simulink model "solar_tracker_plant"  (R2026b)
settings: Solver=ode4  StopTime=60  FixedStep=0.01
model workspace (MAT data in the model file):
  targetAzimuthInput = timeseries
  targetAzimuthInput.Name = 'unnamed'
  targetAzimuthInput.DataInfo = tsdata.datametadata
  targetAzimuthInput.DataInfo.Interpolation = tsdata.interpolation
  targetAzimuthInput.DataInfo.Interpolation.Fhandle : function handle (value not decoded)
  targetAzimuthInput.DataInfo.Interpolation.Name = 'linear'
  targetAzimuthInput.TimeInfo = tsdata.timemetadata
  targetAzimuthInput.TimeInfo.Length = 2
  targetAzimuthInput.TimeInfo.DuplicateTimes = 0
  targetAzimuthInput.TimeInfo.Time_ = [0; 86400]
  targetAzimuthInput.TimeInfo.Initialized = 1
  targetAzimuthInput.QualityInfo = tsdata.qualmetadata
  targetAzimuthInput.Data_ = [0; 0]
  targetTiltInput = timeseries
  targetTiltInput.Name = 'unnamed'
  targetTiltInput.DataInfo = tsdata.datametadata
  targetTiltInput.DataInfo.Interpolation = tsdata.interpolation
  targetTiltInput.DataInfo.Interpolation.Fhandle : function handle (value not decoded)
  targetTiltInput.DataInfo.Interpolation.Name = 'linear'
  targetTiltInput.TimeInfo = tsdata.timemetadata
  targetTiltInput.TimeInfo.Length = 2
  targetTiltInput.TimeInfo.DuplicateTimes = 0
  targetTiltInput.TimeInfo.Time_ = [0; 86400]
  targetTiltInput.TimeInfo.Initialized = 1
  targetTiltInput.QualityInfo = tsdata.qualmetadata
  targetTiltInput.Data_ = [0; 0]
libraries: fl_lib x22, nesl_utility x16, sl_discontinuities x2
settings Model: Creator=Jhons Janner Samuel  LastModifiedBy=Jhons Janner Samuel
settings SimscapeCC: SimscapeLogType=all  SimscapeNominalValues="[{\"value\":\"1\",\"unit\":\"A\"},{\"value\":\"1\",\"unit\":\"bar\"},{\"value\":\"1\",\"unit\":\"cm^2\"},{\"value\":\"1\",\"unit\":\"cm^3/s\"},{\"value\":\"1\",\"unit\":\"kJ/kg\"},{\"value\":\"1\",\"unit\":\"kW\"},{\"value\":\"1\",\"unit\":\"l\"},{\"value\":\"1\",\"unit\":\"N\"},{\"value\":\"1\",\"unit\":\"N*m\"},{\"value\":\"1\",\"unit\":\"V\"},{\"value\":\"0.001\",\"unit\":\"Wb\"}]"  SimscapeUseEnergyAccounting=off

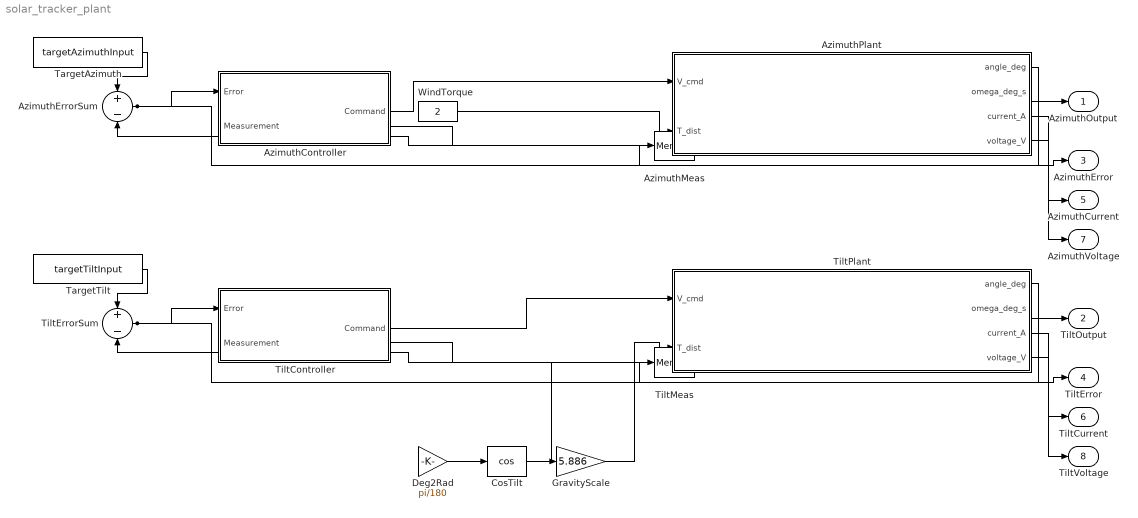
== system solar_tracker_plant ==
  AzimuthController : Subsystem
  AzimuthErrorSum : Sum  Inputs=+-
  AzimuthMeas : Memory
  AzimuthPlant : Subsystem
  CosTilt : Trigonometry  Operator=cos
  Deg2Rad : Gain  Gain=pi/180
  GravityScale : Gain  Gain=5.886
  TargetAzimuth : FromWorkspace  VariableName=targetAzimuthInput
  TargetTilt : FromWorkspace  VariableName=targetTiltInput
  TiltController : Subsystem
  TiltErrorSum : Sum  Inputs=+-
  TiltMeas : Memory
  TiltPlant : Subsystem
  WindTorque : Constant  Value=2
  AzimuthOutput : Outport
  TiltOutput : Outport  Port=2
  AzimuthError : Outport  Port=3
  TiltError : Outport  Port=4
  AzimuthCurrent : Outport  Port=5
  TiltCurrent : Outport  Port=6
  AzimuthVoltage : Outport  Port=7
  TiltVoltage : Outport  Port=8
  wires:
  TargetAzimuth/1 -> AzimuthErrorSum/1
  TargetTilt/1 -> TiltErrorSum/1
  TiltMeas/1 -> Deg2Rad/1, TiltOutput/1, TiltErrorSum/2, TiltController/2(Measurement)
  Deg2Rad/1 -> CosTilt/1
  CosTilt/1 -> GravityScale/1
  AzimuthErrorSum/1 -> AzimuthController/1(Error), AzimuthError/1
  AzimuthController/1(Command) -> AzimuthPlant/1(V_cmd)
  AzimuthPlant/1(angle_deg) -> AzimuthMeas/1
  AzimuthMeas/1 -> AzimuthOutput/1, AzimuthErrorSum/2, AzimuthController/2(Measurement)
  TiltErrorSum/1 -> TiltController/1(Error), TiltError/1
  TiltController/1(Command) -> TiltPlant/1(V_cmd)
  TiltPlant/1(angle_deg) -> TiltMeas/1
  AzimuthPlant/3(current_A) -> AzimuthCurrent/1
  TiltPlant/3(current_A) -> TiltCurrent/1
  AzimuthPlant/4(voltage_V) -> AzimuthVoltage/1
  TiltPlant/4(voltage_V) -> TiltVoltage/1
  WindTorque/1 -> AzimuthPlant/2(T_dist)
  GravityScale/1 -> TiltPlant/2(T_dist)

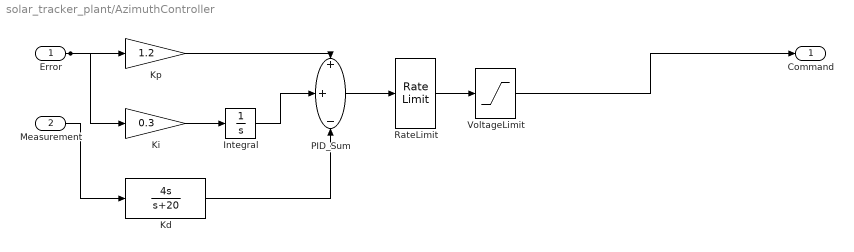
== system solar_tracker_plant/AzimuthController ==
  Error : Inport
  Measurement : Inport  Port=2
  Integral : Integrator  LimitOutput=on  UpperSaturationLimit=80  LowerSaturationLimit=-80
  Kd : TransferFcn  Numerator=[4 0]  Denominator=[1 20]
  Ki : Gain  Gain=0.3
  Kp : Gain  Gain=1.2
  PID_Sum : Sum  Inputs=++-
  RateLimit : RateLimiter  RisingSlewLimit=2400  FallingSlewLimit=-2400  SampleTimeMode=inherited
  VoltageLimit : Saturate  UpperLimit=24  LowerLimit=-24
  Command : Outport
  wires:
  Error/1 -> Kp/1, Ki/1
  Ki/1 -> Integral/1
  Measurement/1 -> Kd/1
  Kp/1 -> PID_Sum/1
  Integral/1 -> PID_Sum/2
  Kd/1 -> PID_Sum/3
  PID_Sum/1 -> RateLimit/1
  RateLimit/1 -> VoltageLimit/1
  VoltageLimit/1 -> Command/1

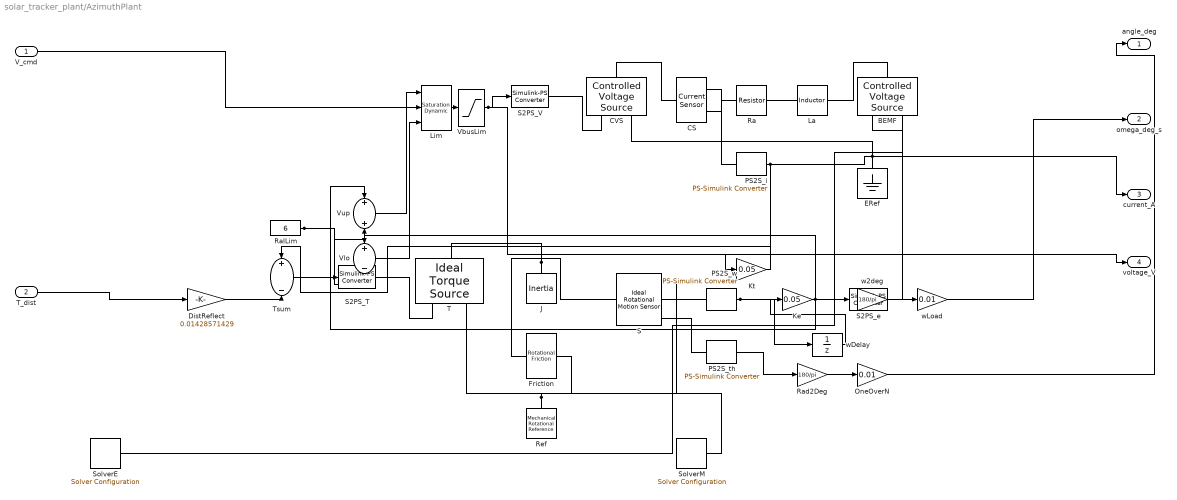
== system solar_tracker_plant/AzimuthPlant ==
  V_cmd : Inport
  T_dist : Inport  Port=2
  BEMF : fl_lib/Electrical/Electrical Sources/Controlled Voltage Source
  CS : fl_lib/Electrical/Electrical Sensors/Current Sensor
  CVS : fl_lib/Electrical/Electrical Sources/Controlled Voltage Source
  DistReflect : Gain  Gain=0.01428571429
  ERef : fl_lib/Electrical/Electrical Elements/Electrical Reference
  Friction : fl_lib/Mechanical/Rotational Elements/Rotational Friction  brkwy_trq=0.01 N*m  brkwy_vel=0.01 rad/s  Col_trq=0.01 N*m  visc_coef=0.0001 N*m*s/rad  w_specify=off  w_priority=None  w=0 rad/s  w_nominal_specify=off  w_nominal_value=1  w_nominal_unit=rad/s  t_specify=off  t_priority=None  t=0 N*m  t_nominal_specify=off  t_nominal_value=1  t_nominal_unit=N*m
  J : fl_lib/Mechanical/Rotational Elements/Inertia  inertia=0.00081 kg*m^2  num_ports=foundation.enum.numPorts2.one  w_specify=off  w_priority=High  w=0 rad/s  w_nominal_specify=off  w_nominal_value=1  w_nominal_unit=rad/s  t_specify=off  t_priority=None  t=0 N*m  t_nominal_specify=off  t_nominal_value=1  t_nominal_unit=N*m
  Ke : Gain  Gain=0.05
  Kt : Gain  Gain=0.05
  La : fl_lib/Electrical/Electrical Elements/Inductor  l=0.0005 H  r=0 Ohm  g=1e-9 1/Ohm  i_specify=off  i_priority=None  i=0 A  i_nominal_specify=off  i_nominal_value=1  i_nominal_unit=A  v_specify=off  v_priority=None  v=0 V  v_nominal_specify=off  v_nominal_value=1  v_nominal_unit=V  i_L_specify=off  i_L_priority=High  i_L=0 A  i_L_nominal_specify=off  i_L_nominal_value=1  i_L_nominal_unit=A
  Lim : sl_discontinuities/Saturation Dynamic  OutMin=[]  OutMax=[]  OutDataTypeStr=Inherit: Same as second input  OutDataType=fixdt(1, 16)  OutScaling=2^-10  DoSatur=off
      settings: LibrarySourceBlock=|
      | simulink/Discontinuities/Saturation
      | Dynamic
  OneOverN : Gain  Gain=0.01
  PS2S_i : nesl_utility/PS-Simulink Converter  PhysicalDomain=network_engine_domain  SubClassName=ps_output  LeftPortType=input  RightPortType=output  PseudoPeriodic=off  Frequencies=[]  VectorFormat=inherit  Unit=inherit  AffineConversion=off
  PS2S_th : nesl_utility/PS-Simulink Converter  PhysicalDomain=network_engine_domain  SubClassName=ps_output  LeftPortType=input  RightPortType=output  PseudoPeriodic=off  Frequencies=[]  VectorFormat=inherit  Unit=inherit  AffineConversion=off
  PS2S_w : nesl_utility/PS-Simulink Converter  PhysicalDomain=network_engine_domain  SubClassName=ps_output  LeftPortType=input  RightPortType=output  PseudoPeriodic=off  Frequencies=[]  VectorFormat=inherit  Unit=inherit  AffineConversion=off
  Ra : fl_lib/Electrical/Electrical Elements/Resistor  R=1.2 Ohm  i_specify=off  i_priority=None  i=0 A  i_nominal_specify=off  i_nominal_value=1  i_nominal_unit=A  v_specify=off  v_priority=None  v=0 V  v_nominal_specify=off  v_nominal_value=1  v_nominal_unit=V
  RaILim : Constant  Value=6
  Rad2Deg : Gain  Gain=180/pi
  Ref : fl_lib/Mechanical/Rotational Elements/Mechanical Rotational Reference
  S : fl_lib/Mechanical/Mechanical Sensors/Ideal Rotational Motion Sensor  reference=foundation.enum.MeasurementReference.difference  acceleration_port=false  velocity_port=true  position_port=true  wrap_angle=false  offset=0 rad
  S2PS_T : nesl_utility/Simulink-PS Converter  PhysicalDomain=network_engine_domain  SubClassName=ps_input  LeftPortType=input  RightPortType=output  PseudoPeriodic=off  Frequencies=[]  NoiseDistribution=none  NoiseParameters=[]  Unit=1  AffineConversion=off  FilteringAndDerivatives=provide  SimscapeFilterOrder=1  InputFilterTimeConstant=0.001  UdotUserProvided=0
  S2PS_V : nesl_utility/Simulink-PS Converter  PhysicalDomain=network_engine_domain  SubClassName=ps_input  LeftPortType=input  RightPortType=output  PseudoPeriodic=off  Frequencies=[]  NoiseDistribution=none  NoiseParameters=[]  Unit=1  AffineConversion=off  FilteringAndDerivatives=provide  SimscapeFilterOrder=1  InputFilterTimeConstant=0.001  UdotUserProvided=0
  S2PS_e : nesl_utility/Simulink-PS Converter  PhysicalDomain=network_engine_domain  SubClassName=ps_input  LeftPortType=input  RightPortType=output  PseudoPeriodic=off  Frequencies=[]  NoiseDistribution=none  NoiseParameters=[]  Unit=1  AffineConversion=off  FilteringAndDerivatives=provide  SimscapeFilterOrder=1  InputFilterTimeConstant=0.001  UdotUserProvided=0
  SolverE : nesl_utility/Solver Configuration  PhysicalDomain=network_engine_domain  SubClassName=solver  LeftPortType=input  RightPortType=generic  Tones=[]  Harmonics=[]  SimulateNoise=off  Profile=off  UseLocalSampling=off  EnableSwitchedLinearOptims=on  FrequencyDomain=off  UseCCode=off  RelTol=0.001  AbsTol=0.001  MinStep=1e-09  ToWorkspace=off  RevertToSquareIcSolve=off  NumHomotopyIterations=100  PhasorMode=off  PhasorModeNumHarmonics=1  ConsistencySolver=NEWTON_XTOL_AFTER_FTOL  CanonicalOrdering=CANONICAL  OptimizeIntermediates=OPTIMIZED  MulticoreSolverChoice=BACKWARD_EULER  IndexReductionMethod=DerivativeReplacement  DoDC=off  ResidualTolerance=1e-09  ConsistencyTolSource=GLOBAL  ConsistencyAbsTol=0.001  ConsistencyRelTol=0.001  ConsistencyTolFactor=0.001  UseLocalSolver=on  LocalSolverChoice=NE_BACKWARD_EULER_ADVANCER  ResolveIndetEquations=on  FunctionEvalNumThread=1  LocalSolverSampleTime=0.01  DoFixedCost=off  MaxNonlinIter=3  MaxModeIter=2  ComputeImpulses=off  ImpulseIterations=2  LinearAlgebra=auto  LinearAlgebraNumThread=0  EquationFormulation=NE_TIME_EF  DelaysMemoryBudget=1024  AutomaticFiltering=on  FilteringTimeConstant=0.001  PartitionStorageMethod=AS_NEEDED  PartitionMemoryBudget=1024  PartitionMethod=BALANCED  MultibodyUseLocalSolver=off  MultibodyLocalSolverChoice=ODE1  MultibodyLocalSolverSampleTime=0.001
  SolverM : nesl_utility/Solver Configuration  PhysicalDomain=network_engine_domain  SubClassName=solver  LeftPortType=input  RightPortType=generic  Tones=[]  Harmonics=[]  SimulateNoise=off  Profile=off  UseLocalSampling=off  EnableSwitchedLinearOptims=on  FrequencyDomain=off  UseCCode=off  RelTol=0.001  AbsTol=0.001  MinStep=1e-09  ToWorkspace=off  RevertToSquareIcSolve=off  NumHomotopyIterations=100  PhasorMode=off  PhasorModeNumHarmonics=1  ConsistencySolver=NEWTON_XTOL_AFTER_FTOL  CanonicalOrdering=CANONICAL  OptimizeIntermediates=OPTIMIZED  MulticoreSolverChoice=BACKWARD_EULER  IndexReductionMethod=DerivativeReplacement  DoDC=off  ResidualTolerance=1e-09  ConsistencyTolSource=GLOBAL  ConsistencyAbsTol=0.001  ConsistencyRelTol=0.001  ConsistencyTolFactor=0.001  UseLocalSolver=on  LocalSolverChoice=NE_BACKWARD_EULER_ADVANCER  ResolveIndetEquations=on  FunctionEvalNumThread=1  LocalSolverSampleTime=0.01  DoFixedCost=off  MaxNonlinIter=3  MaxModeIter=2  ComputeImpulses=off  ImpulseIterations=2  LinearAlgebra=auto  LinearAlgebraNumThread=0  EquationFormulation=NE_TIME_EF  DelaysMemoryBudget=1024  AutomaticFiltering=on  FilteringTimeConstant=0.001  PartitionStorageMethod=AS_NEEDED  PartitionMemoryBudget=1024  PartitionMethod=BALANCED  MultibodyUseLocalSolver=off  MultibodyLocalSolverChoice=ODE1  MultibodyLocalSolverSampleTime=0.001
  T : fl_lib/Mechanical/Mechanical Sources/Ideal Torque Source
  Tsum : Sum  Inputs=+-
  VbusLim : Saturate  UpperLimit=24  LowerLimit=-24
  Vlo : Sum  Inputs=+-
  Vup : Sum
  w2deg : Gain  Gain=180/pi
  wDelay : UnitDelay  SampleTime=0.01
  wLoad : Gain  Gain=0.01
  angle_deg : Outport
  omega_deg_s : Outport  Port=2
  current_A : Outport  Port=3
  voltage_V : Outport  Port=4
  wires:
  V_cmd/1 -> Lim/2
  Vup/1 -> Lim/1
  Vlo/1 -> Lim/3
  Lim/1 -> VbusLim/1
  VbusLim/1 -> S2PS_V/1, voltage_V/1
  Ke/1 -> Vup/1, Vlo/1, S2PS_e/1
  RaILim/1 -> Vup/2, Vlo/2
  PS2S_i/1 -> Kt/1, current_A/1
  Kt/1 -> Tsum/1
  T_dist/1 -> DistReflect/1
  DistReflect/1 -> Tsum/2
  Tsum/1 -> S2PS_T/1
  PS2S_w/1 -> wDelay/1, w2deg/1
  wDelay/1 -> Ke/1
  w2deg/1 -> wLoad/1
  wLoad/1 -> omega_deg_s/1
  PS2S_th/1 -> Rad2Deg/1
  Rad2Deg/1 -> OneOverN/1
  OneOverN/1 -> angle_deg/1
  connections:
  CS/RConn1 -- PS2S_i/LConn1
  S2PS_V/RConn1 -- CVS/RConn1
  S2PS_e/RConn1 -- BEMF/RConn1
  S2PS_T/RConn1 -- T/RConn1
  CVS/LConn1 -- CS/LConn1
  CS/RConn2 -- Ra/LConn1
  Ra/RConn1 -- La/LConn1
  La/RConn1 -- BEMF/LConn1
  BEMF/RConn2 -- CVS/RConn2 -- ERef/LConn1 -- SolverE/RConn1
  T/LConn1 -- Friction/LConn1 -- J/LConn1 -- S/LConn1
  Friction/RConn1 -- T/RConn2 -- S/RConn1 -- Ref/LConn1 -- SolverM/RConn1
  S/RConn2 -- PS2S_w/LConn1
  S/RConn3 -- PS2S_th/LConn1

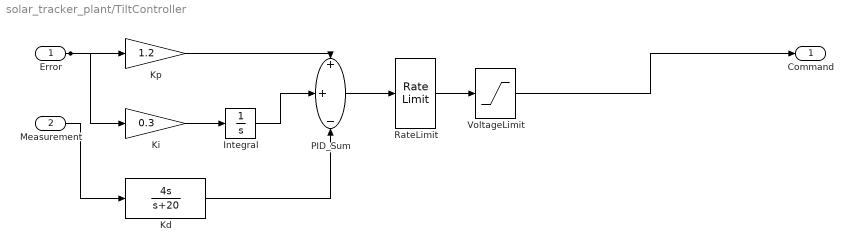
== system solar_tracker_plant/TiltController ==
  Error : Inport
  Measurement : Inport  Port=2
  Integral : Integrator  LimitOutput=on  UpperSaturationLimit=80  LowerSaturationLimit=-80
  Kd : TransferFcn  Numerator=[4 0]  Denominator=[1 20]
  Ki : Gain  Gain=0.3
  Kp : Gain  Gain=1.2
  PID_Sum : Sum  Inputs=++-
  RateLimit : RateLimiter  RisingSlewLimit=2400  FallingSlewLimit=-2400  SampleTimeMode=inherited
  VoltageLimit : Saturate  UpperLimit=24  LowerLimit=-24
  Command : Outport
  wires:
  Error/1 -> Kp/1, Ki/1
  Ki/1 -> Integral/1
  Measurement/1 -> Kd/1
  Kp/1 -> PID_Sum/1
  Integral/1 -> PID_Sum/2
  Kd/1 -> PID_Sum/3
  PID_Sum/1 -> RateLimit/1
  RateLimit/1 -> VoltageLimit/1
  VoltageLimit/1 -> Command/1

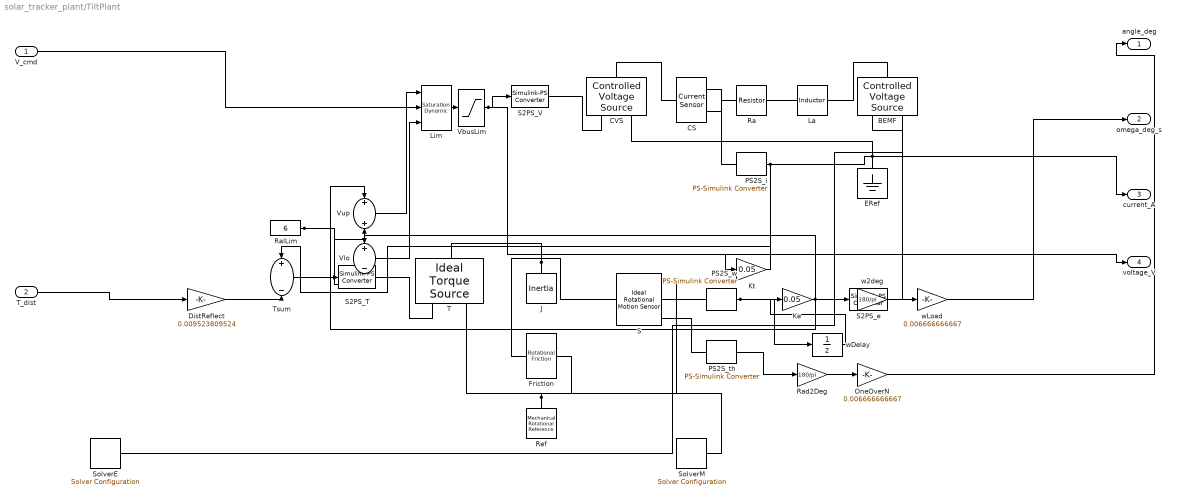
== system solar_tracker_plant/TiltPlant ==
  V_cmd : Inport
  T_dist : Inport  Port=2
  BEMF : fl_lib/Electrical/Electrical Sources/Controlled Voltage Source
  CS : fl_lib/Electrical/Electrical Sensors/Current Sensor
  CVS : fl_lib/Electrical/Electrical Sources/Controlled Voltage Source
  DistReflect : Gain  Gain=0.009523809524
  ERef : fl_lib/Electrical/Electrical Elements/Electrical Reference
  Friction : fl_lib/Mechanical/Rotational Elements/Rotational Friction  brkwy_trq=0.01 N*m  brkwy_vel=0.01 rad/s  Col_trq=0.01 N*m  visc_coef=0.0001 N*m*s/rad  w_specify=off  w_priority=None  w=0 rad/s  w_nominal_specify=off  w_nominal_value=1  w_nominal_unit=rad/s  t_specify=off  t_priority=None  t=0 N*m  t_nominal_specify=off  t_nominal_value=1  t_nominal_unit=N*m
  J : fl_lib/Mechanical/Rotational Elements/Inertia  inertia=0.0001655555556 kg*m^2  num_ports=foundation.enum.numPorts2.one  w_specify=off  w_priority=High  w=0 rad/s  w_nominal_specify=off  w_nominal_value=1  w_nominal_unit=rad/s  t_specify=off  t_priority=None  t=0 N*m  t_nominal_specify=off  t_nominal_value=1  t_nominal_unit=N*m
  Ke : Gain  Gain=0.05
  Kt : Gain  Gain=0.05
  La : fl_lib/Electrical/Electrical Elements/Inductor  l=0.0005 H  r=0 Ohm  g=1e-9 1/Ohm  i_specify=off  i_priority=None  i=0 A  i_nominal_specify=off  i_nominal_value=1  i_nominal_unit=A  v_specify=off  v_priority=None  v=0 V  v_nominal_specify=off  v_nominal_value=1  v_nominal_unit=V  i_L_specify=off  i_L_priority=High  i_L=0 A  i_L_nominal_specify=off  i_L_nominal_value=1  i_L_nominal_unit=A
  Lim : sl_discontinuities/Saturation Dynamic  OutMin=[]  OutMax=[]  OutDataTypeStr=Inherit: Same as second input  OutDataType=fixdt(1, 16)  OutScaling=2^-10  DoSatur=off
      settings: LibrarySourceBlock=|
      | simulink/Discontinuities/Saturation
      | Dynamic
  OneOverN : Gain  Gain=0.006666666667
  PS2S_i : nesl_utility/PS-Simulink Converter  PhysicalDomain=network_engine_domain  SubClassName=ps_output  LeftPortType=input  RightPortType=output  PseudoPeriodic=off  Frequencies=[]  VectorFormat=inherit  Unit=inherit  AffineConversion=off
  PS2S_th : nesl_utility/PS-Simulink Converter  PhysicalDomain=network_engine_domain  SubClassName=ps_output  LeftPortType=input  RightPortType=output  PseudoPeriodic=off  Frequencies=[]  VectorFormat=inherit  Unit=inherit  AffineConversion=off
  PS2S_w : nesl_utility/PS-Simulink Converter  PhysicalDomain=network_engine_domain  SubClassName=ps_output  LeftPortType=input  RightPortType=output  PseudoPeriodic=off  Frequencies=[]  VectorFormat=inherit  Unit=inherit  AffineConversion=off
  Ra : fl_lib/Electrical/Electrical Elements/Resistor  R=1.2 Ohm  i_specify=off  i_priority=None  i=0 A  i_nominal_specify=off  i_nominal_value=1  i_nominal_unit=A  v_specify=off  v_priority=None  v=0 V  v_nominal_specify=off  v_nominal_value=1  v_nominal_unit=V
  RaILim : Constant  Value=6
  Rad2Deg : Gain  Gain=180/pi
  Ref : fl_lib/Mechanical/Rotational Elements/Mechanical Rotational Reference
  S : fl_lib/Mechanical/Mechanical Sensors/Ideal Rotational Motion Sensor  reference=foundation.enum.MeasurementReference.difference  acceleration_port=false  velocity_port=true  position_port=true  wrap_angle=false  offset=0 rad
  S2PS_T : nesl_utility/Simulink-PS Converter  PhysicalDomain=network_engine_domain  SubClassName=ps_input  LeftPortType=input  RightPortType=output  PseudoPeriodic=off  Frequencies=[]  NoiseDistribution=none  NoiseParameters=[]  Unit=1  AffineConversion=off  FilteringAndDerivatives=provide  SimscapeFilterOrder=1  InputFilterTimeConstant=0.001  UdotUserProvided=0
  S2PS_V : nesl_utility/Simulink-PS Converter  PhysicalDomain=network_engine_domain  SubClassName=ps_input  LeftPortType=input  RightPortType=output  PseudoPeriodic=off  Frequencies=[]  NoiseDistribution=none  NoiseParameters=[]  Unit=1  AffineConversion=off  FilteringAndDerivatives=provide  SimscapeFilterOrder=1  InputFilterTimeConstant=0.001  UdotUserProvided=0
  S2PS_e : nesl_utility/Simulink-PS Converter  PhysicalDomain=network_engine_domain  SubClassName=ps_input  LeftPortType=input  RightPortType=output  PseudoPeriodic=off  Frequencies=[]  NoiseDistribution=none  NoiseParameters=[]  Unit=1  AffineConversion=off  FilteringAndDerivatives=provide  SimscapeFilterOrder=1  InputFilterTimeConstant=0.001  UdotUserProvided=0
  SolverE : nesl_utility/Solver Configuration  PhysicalDomain=network_engine_domain  SubClassName=solver  LeftPortType=input  RightPortType=generic  Tones=[]  Harmonics=[]  SimulateNoise=off  Profile=off  UseLocalSampling=off  EnableSwitchedLinearOptims=on  FrequencyDomain=off  UseCCode=off  RelTol=0.001  AbsTol=0.001  MinStep=1e-09  ToWorkspace=off  RevertToSquareIcSolve=off  NumHomotopyIterations=100  PhasorMode=off  PhasorModeNumHarmonics=1  ConsistencySolver=NEWTON_XTOL_AFTER_FTOL  CanonicalOrdering=CANONICAL  OptimizeIntermediates=OPTIMIZED  MulticoreSolverChoice=BACKWARD_EULER  IndexReductionMethod=DerivativeReplacement  DoDC=off  ResidualTolerance=1e-09  ConsistencyTolSource=GLOBAL  ConsistencyAbsTol=0.001  ConsistencyRelTol=0.001  ConsistencyTolFactor=0.001  UseLocalSolver=on  LocalSolverChoice=NE_BACKWARD_EULER_ADVANCER  ResolveIndetEquations=on  FunctionEvalNumThread=1  LocalSolverSampleTime=0.01  DoFixedCost=off  MaxNonlinIter=3  MaxModeIter=2  ComputeImpulses=off  ImpulseIterations=2  LinearAlgebra=auto  LinearAlgebraNumThread=0  EquationFormulation=NE_TIME_EF  DelaysMemoryBudget=1024  AutomaticFiltering=on  FilteringTimeConstant=0.001  PartitionStorageMethod=AS_NEEDED  PartitionMemoryBudget=1024  PartitionMethod=BALANCED  MultibodyUseLocalSolver=off  MultibodyLocalSolverChoice=ODE1  MultibodyLocalSolverSampleTime=0.001
  SolverM : nesl_utility/Solver Configuration  PhysicalDomain=network_engine_domain  SubClassName=solver  LeftPortType=input  RightPortType=generic  Tones=[]  Harmonics=[]  SimulateNoise=off  Profile=off  UseLocalSampling=off  EnableSwitchedLinearOptims=on  FrequencyDomain=off  UseCCode=off  RelTol=0.001  AbsTol=0.001  MinStep=1e-09  ToWorkspace=off  RevertToSquareIcSolve=off  NumHomotopyIterations=100  PhasorMode=off  PhasorModeNumHarmonics=1  ConsistencySolver=NEWTON_XTOL_AFTER_FTOL  CanonicalOrdering=CANONICAL  OptimizeIntermediates=OPTIMIZED  MulticoreSolverChoice=BACKWARD_EULER  IndexReductionMethod=DerivativeReplacement  DoDC=off  ResidualTolerance=1e-09  ConsistencyTolSource=GLOBAL  ConsistencyAbsTol=0.001  ConsistencyRelTol=0.001  ConsistencyTolFactor=0.001  UseLocalSolver=on  LocalSolverChoice=NE_BACKWARD_EULER_ADVANCER  ResolveIndetEquations=on  FunctionEvalNumThread=1  LocalSolverSampleTime=0.01  DoFixedCost=off  MaxNonlinIter=3  MaxModeIter=2  ComputeImpulses=off  ImpulseIterations=2  LinearAlgebra=auto  LinearAlgebraNumThread=0  EquationFormulation=NE_TIME_EF  DelaysMemoryBudget=1024  AutomaticFiltering=on  FilteringTimeConstant=0.001  PartitionStorageMethod=AS_NEEDED  PartitionMemoryBudget=1024  PartitionMethod=BALANCED  MultibodyUseLocalSolver=off  MultibodyLocalSolverChoice=ODE1  MultibodyLocalSolverSampleTime=0.001
  T : fl_lib/Mechanical/Mechanical Sources/Ideal Torque Source
  Tsum : Sum  Inputs=+-
  VbusLim : Saturate  UpperLimit=24  LowerLimit=-24
  Vlo : Sum  Inputs=+-
  Vup : Sum
  w2deg : Gain  Gain=180/pi
  wDelay : UnitDelay  SampleTime=0.01
  wLoad : Gain  Gain=0.006666666667
  angle_deg : Outport
  omega_deg_s : Outport  Port=2
  current_A : Outport  Port=3
  voltage_V : Outport  Port=4
  wires:
  V_cmd/1 -> Lim/2
  Vup/1 -> Lim/1
  Vlo/1 -> Lim/3
  Lim/1 -> VbusLim/1
  VbusLim/1 -> S2PS_V/1, voltage_V/1
  Ke/1 -> Vup/1, Vlo/1, S2PS_e/1
  RaILim/1 -> Vup/2, Vlo/2
  PS2S_i/1 -> Kt/1, current_A/1
  Kt/1 -> Tsum/1
  T_dist/1 -> DistReflect/1
  DistReflect/1 -> Tsum/2
  Tsum/1 -> S2PS_T/1
  PS2S_w/1 -> wDelay/1, w2deg/1
  wDelay/1 -> Ke/1
  w2deg/1 -> wLoad/1
  wLoad/1 -> omega_deg_s/1
  PS2S_th/1 -> Rad2Deg/1
  Rad2Deg/1 -> OneOverN/1
  OneOverN/1 -> angle_deg/1
  connections:
  CS/RConn1 -- PS2S_i/LConn1
  S2PS_V/RConn1 -- CVS/RConn1
  S2PS_e/RConn1 -- BEMF/RConn1
  S2PS_T/RConn1 -- T/RConn1
  CVS/LConn1 -- CS/LConn1
  CS/RConn2 -- Ra/LConn1
  Ra/RConn1 -- La/LConn1
  La/RConn1 -- BEMF/LConn1
  BEMF/RConn2 -- CVS/RConn2 -- ERef/LConn1 -- SolverE/RConn1
  T/LConn1 -- Friction/LConn1 -- J/LConn1 -- S/LConn1
  Friction/RConn1 -- T/RConn2 -- S/RConn1 -- Ref/LConn1 -- SolverM/RConn1
  S/RConn2 -- PS2S_w/LConn1
  S/RConn3 -- PS2S_th/LConn1
